simulink model "EV_Bus_Forward_before_noise_update"  (R2025a)
settings: Solver=ode23t  StartTime=0.0  StopTime=300  MaxStep=0.01  RelTol=1e-5  AbsTol=1e-7
model workspace (MAT data in the model file):
  Comp : object (value not decoded)
  MeasuredForceBias = 1114.3044183
  MeasuredTraction = [0 0.01 0.02 0.03 0.04 0.05 0.06 0.07 0.08 0.09 0.1 0.11 ... (60002 elements, 30001x2)]
  P : object (value not decoded)
  SignalNames : object (value not decoded)
  SlopeProfile = [0 85 100 140 155 180 200 300 0 0 4 4 ... (16 elements, 8x2)]
  SpeedProfile = [0 5 25 55 70 85 105 140 160 180 200 225 ... (32 elements, 16x2)]
  TemperatureProfile = [0  25; 150  30; 300  35]
values from neighbouring files (symbols this model uses):
  P =     [EV_Bus_parameters.mat]
symbols that are objects in the model workspace (value not decoded): Comp
(part 2 of 2)

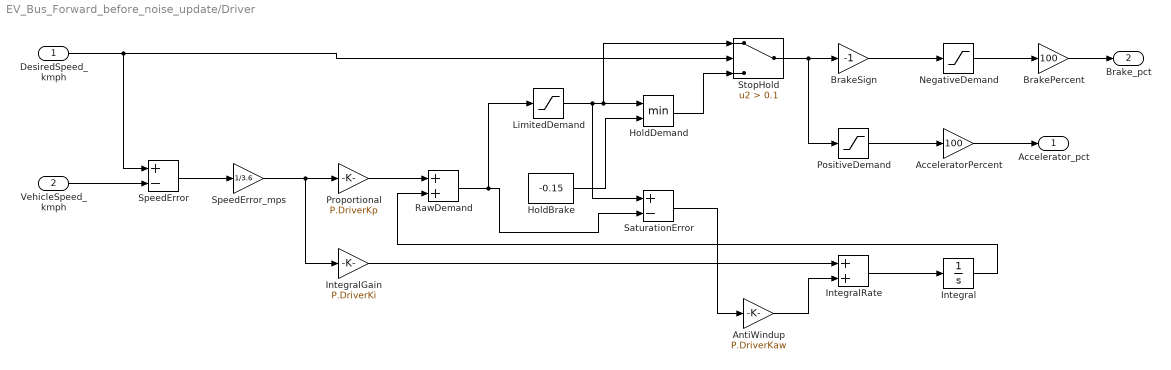
== system EV_Bus_Forward_before_noise_update/Driver ==
  DesiredSpeed_kmph : Inport
  VehicleSpeed_kmph : Inport  Port=2
  AcceleratorPercent : Gain  Gain=100
  AntiWindup : Gain  Gain=P.DriverKaw
  BrakePercent : Gain  Gain=100
  BrakeSign : Gain  Gain=-1
  HoldBrake : Constant  Value=-0.15
  HoldDemand : MinMax  Inputs=2
  Integral : Integrator  LimitOutput=on  UpperSaturationLimit=0.6  LowerSaturationLimit=-0.6
  IntegralGain : Gain  Gain=P.DriverKi
  IntegralRate : Sum
  LimitedDemand : Saturate  UpperLimit=1  LowerLimit=-1
  NegativeDemand : Saturate  UpperLimit=1  LowerLimit=0
  PositiveDemand : Saturate  UpperLimit=1  LowerLimit=0
  Proportional : Gain  Gain=P.DriverKp
  RawDemand : Sum
  SaturationError : Sum  Inputs=+-
  SpeedError : Sum  Inputs=+-
  SpeedError_mps : Gain  Gain=1/3.6
  StopHold : Switch  Criteria=u2 > Threshold  Threshold=0.1  SaturateOnIntegerOverflow=off  InputSameDT=off
  Accelerator_pct : Outport
  Brake_pct : Outport  Port=2
  wires:
  BrakePercent/1 -> Brake_pct/1
  NegativeDemand/1 -> BrakePercent/1
  BrakeSign/1 -> NegativeDemand/1
  AcceleratorPercent/1 -> Accelerator_pct/1
  PositiveDemand/1 -> AcceleratorPercent/1
  StopHold/1 -> PositiveDemand/1, BrakeSign/1
  HoldDemand/1 -> StopHold/3
  HoldBrake/1 -> HoldDemand/2
  IntegralRate/1 -> Integral/1
  AntiWindup/1 -> IntegralRate/2
  IntegralGain/1 -> IntegralRate/1
  SaturationError/1 -> AntiWindup/1
  LimitedDemand/1 -> HoldDemand/1, StopHold/1, SaturationError/1
  RawDemand/1 -> LimitedDemand/1, SaturationError/2
  Integral/1 -> RawDemand/2
  Proportional/1 -> RawDemand/1
  SpeedError_mps/1 -> Proportional/1, IntegralGain/1
  SpeedError/1 -> SpeedError_mps/1
  VehicleSpeed_kmph/1 -> SpeedError/2
  DesiredSpeed_kmph/1 -> SpeedError/1, StopHold/2

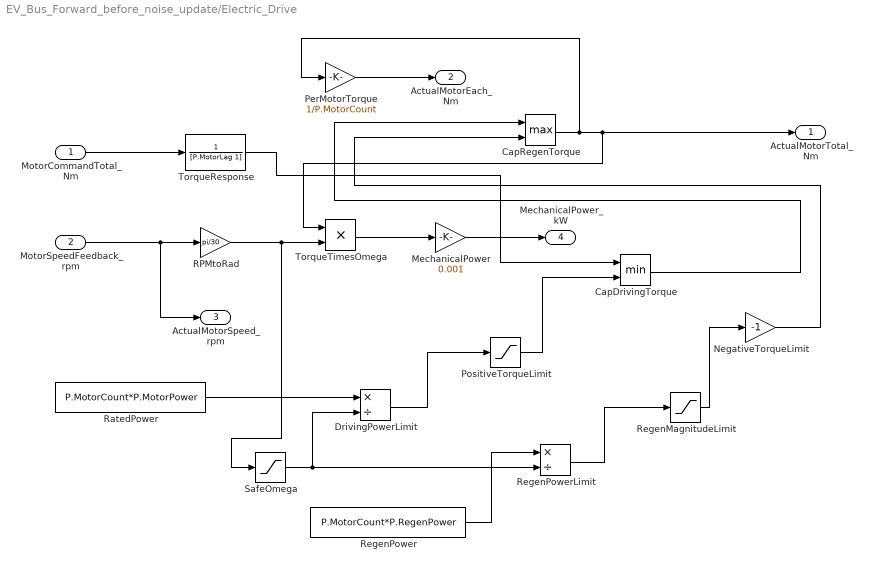
== system EV_Bus_Forward_before_noise_update/Electric_Drive ==
  MotorCommandTotal_Nm : Inport
  MotorSpeedFeedback_rpm : Inport  Port=2
  CapDrivingTorque : MinMax  Inputs=2
  CapRegenTorque : MinMax  Function=max  Inputs=2
  DrivingPowerLimit : Product  Inputs=*/
  MechanicalPower : Gain  Gain=0.001
  NegativeTorqueLimit : Gain  Gain=-1
  PerMotorTorque : Gain  Gain=1/P.MotorCount
  PositiveTorqueLimit : Saturate  UpperLimit=P.MotorCount*P.MotorPeakTorque  LowerLimit=0
  RPMtoRad : Gain  Gain=pi/30
  RatedPower : Constant  Value=P.MotorCount*P.MotorPower
  RegenMagnitudeLimit : Saturate  UpperLimit=P.MotorCount*P.RegenPeakTorque  LowerLimit=0
  RegenPower : Constant  Value=P.MotorCount*P.RegenPower
  RegenPowerLimit : Product  Inputs=*/
  SafeOmega : Saturate  UpperLimit=inf  LowerLimit=1
  TorqueResponse : TransferFcn  Denominator=[P.MotorLag 1]
  TorqueTimesOmega : Product  Inputs=**
  ActualMotorTotal_Nm : Outport
  ActualMotorEach_Nm : Outport  Port=2
  ActualMotorSpeed_rpm : Outport  Port=3
  MechanicalPower_kW : Outport  Port=4
  wires:
  MechanicalPower/1 -> MechanicalPower_kW/1
  TorqueTimesOmega/1 -> MechanicalPower/1
  MotorSpeedFeedback_rpm/1 -> ActualMotorSpeed_rpm/1, RPMtoRad/1
  PerMotorTorque/1 -> ActualMotorEach_Nm/1
  MotorCommandTotal_Nm/1 -> TorqueResponse/1
  CapRegenTorque/1 -> TorqueTimesOmega/1, ActualMotorTotal_Nm/1, PerMotorTorque/1
  NegativeTorqueLimit/1 -> CapRegenTorque/2
  CapDrivingTorque/1 -> CapRegenTorque/1
  PositiveTorqueLimit/1 -> CapDrivingTorque/2
  RegenMagnitudeLimit/1 -> NegativeTorqueLimit/1
  RegenPowerLimit/1 -> RegenMagnitudeLimit/1
  RegenPower/1 -> RegenPowerLimit/1
  DrivingPowerLimit/1 -> PositiveTorqueLimit/1
  SafeOmega/1 -> RegenPowerLimit/2, DrivingPowerLimit/2
  RatedPower/1 -> DrivingPowerLimit/1
  TorqueResponse/1 -> CapDrivingTorque/1
  RPMtoRad/1 -> SafeOmega/1, TorqueTimesOmega/2

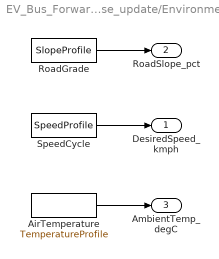
== system EV_Bus_Forward_before_noise_update/Environment ==
  AirTemperature : FromWorkspace  VariableName=TemperatureProfile
  RoadGrade : FromWorkspace  VariableName=SlopeProfile
  SpeedCycle : FromWorkspace  VariableName=SpeedProfile
  DesiredSpeed_kmph : Outport
  RoadSlope_pct : Outport  Port=2
  AmbientTemp_degC : Outport  Port=3
  wires:
  AirTemperature/1 -> AmbientTemp_degC/1
  RoadGrade/1 -> RoadSlope_pct/1
  SpeedCycle/1 -> DesiredSpeed_kmph/1

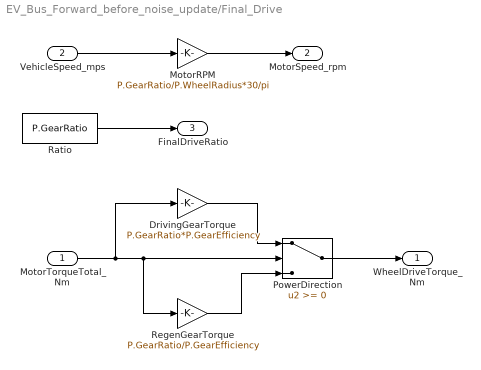
== system EV_Bus_Forward_before_noise_update/Final_Drive ==
  MotorTorqueTotal_Nm : Inport
  VehicleSpeed_mps : Inport  Port=2
  DrivingGearTorque : Gain  Gain=P.GearRatio*P.GearEfficiency
  MotorRPM : Gain  Gain=P.GearRatio/P.WheelRadius*30/pi
  PowerDirection : Switch  SaturateOnIntegerOverflow=off  InputSameDT=off
  Ratio : Constant  Value=P.GearRatio
  RegenGearTorque : Gain  Gain=P.GearRatio/P.GearEfficiency
  WheelDriveTorque_Nm : Outport
  MotorSpeed_rpm : Outport  Port=2
  FinalDriveRatio : Outport  Port=3
  wires:
  Ratio/1 -> FinalDriveRatio/1
  MotorRPM/1 -> MotorSpeed_rpm/1
  VehicleSpeed_mps/1 -> MotorRPM/1
  PowerDirection/1 -> WheelDriveTorque_Nm/1
  RegenGearTorque/1 -> PowerDirection/3
  DrivingGearTorque/1 -> PowerDirection/1
  MotorTorqueTotal_Nm/1 -> PowerDirection/2, RegenGearTorque/1, DrivingGearTorque/1

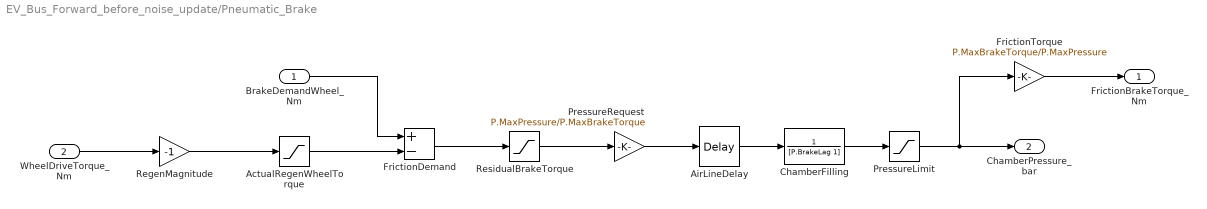
== system EV_Bus_Forward_before_noise_update/Pneumatic_Brake ==
  BrakeDemandWheel_Nm : Inport
  WheelDriveTorque_Nm : Inport  Port=2
  ActualRegenWheelTorque : Saturate  UpperLimit=inf  LowerLimit=0
  AirLineDelay : TransportDelay  DelayTime=P.BrakeDelay
  ChamberFilling : TransferFcn  Denominator=[P.BrakeLag 1]
  FrictionDemand : Sum  Inputs=+-
  FrictionTorque : Gain  Gain=P.MaxBrakeTorque/P.MaxPressure
  PressureLimit : Saturate  UpperLimit=P.MaxPressure  LowerLimit=0
  PressureRequest : Gain  Gain=P.MaxPressure/P.MaxBrakeTorque
  RegenMagnitude : Gain  Gain=-1
  ResidualBrakeTorque : Saturate  UpperLimit=P.MaxBrakeTorque  LowerLimit=0
  FrictionBrakeTorque_Nm : Outport
  ChamberPressure_bar : Outport  Port=2
  wires:
  FrictionTorque/1 -> FrictionBrakeTorque_Nm/1
  PressureLimit/1 -> ChamberPressure_bar/1, FrictionTorque/1
  ChamberFilling/1 -> PressureLimit/1
  AirLineDelay/1 -> ChamberFilling/1
  PressureRequest/1 -> AirLineDelay/1
  ResidualBrakeTorque/1 -> PressureRequest/1
  FrictionDemand/1 -> ResidualBrakeTorque/1
  ActualRegenWheelTorque/1 -> FrictionDemand/2
  BrakeDemandWheel_Nm/1 -> FrictionDemand/1
  RegenMagnitude/1 -> ActualRegenWheelTorque/1
  WheelDriveTorque_Nm/1 -> RegenMagnitude/1

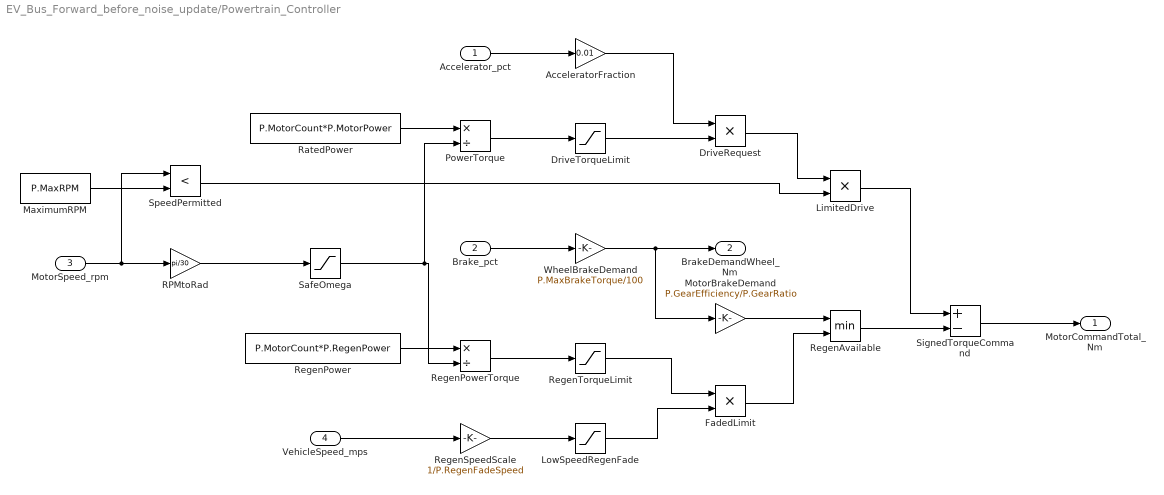
== system EV_Bus_Forward_before_noise_update/Powertrain_Controller ==
  Accelerator_pct : Inport
  Brake_pct : Inport  Port=2
  MotorSpeed_rpm : Inport  Port=3
  VehicleSpeed_mps : Inport  Port=4
  AcceleratorFraction : Gain  Gain=0.01
  DriveRequest : Product  Inputs=**
  DriveTorqueLimit : Saturate  UpperLimit=P.MotorCount*P.MotorPeakTorque  LowerLimit=0
  FadedLimit : Product  Inputs=**
  LimitedDrive : Product  Inputs=**
  LowSpeedRegenFade : Saturate  UpperLimit=1  LowerLimit=0
  MaximumRPM : Constant  Value=P.MaxRPM
  MotorBrakeDemand : Gain  Gain=P.GearEfficiency/P.GearRatio
  PowerTorque : Product  Inputs=*/
  RPMtoRad : Gain  Gain=pi/30
  RatedPower : Constant  Value=P.MotorCount*P.MotorPower
  RegenAvailable : MinMax  Inputs=2
  RegenPower : Constant  Value=P.MotorCount*P.RegenPower
  RegenPowerTorque : Product  Inputs=*/
  RegenSpeedScale : Gain  Gain=1/P.RegenFadeSpeed
  RegenTorqueLimit : Saturate  UpperLimit=P.MotorCount*P.RegenPeakTorque  LowerLimit=0
  SafeOmega : Saturate  UpperLimit=inf  LowerLimit=1
  SignedTorqueCommand : Sum  Inputs=+-
  SpeedPermitted : RelationalOperator  Operator=<  OutDataTypeStr=boolean  RndMeth=Simplest  InputSameDT=off
  WheelBrakeDemand : Gain  Gain=P.MaxBrakeTorque/100
  MotorCommandTotal_Nm : Outport
  BrakeDemandWheel_Nm : Outport  Port=2
  wires:
  SignedTorqueCommand/1 -> MotorCommandTotal_Nm/1
  RegenAvailable/1 -> SignedTorqueCommand/2
  LimitedDrive/1 -> SignedTorqueCommand/1
  SpeedPermitted/1 -> LimitedDrive/2
  DriveRequest/1 -> LimitedDrive/1
  FadedLimit/1 -> RegenAvailable/2
  LowSpeedRegenFade/1 -> FadedLimit/2
  RegenTorqueLimit/1 -> FadedLimit/1
  MotorBrakeDemand/1 -> RegenAvailable/1
  WheelBrakeDemand/1 -> BrakeDemandWheel_Nm/1, MotorBrakeDemand/1
  Brake_pct/1 -> WheelBrakeDemand/1
  MaximumRPM/1 -> SpeedPermitted/2
  DriveTorqueLimit/1 -> DriveRequest/2
  AcceleratorFraction/1 -> DriveRequest/1
  Accelerator_pct/1 -> AcceleratorFraction/1
  RegenSpeedScale/1 -> LowSpeedRegenFade/1
  VehicleSpeed_mps/1 -> RegenSpeedScale/1
  RegenPowerTorque/1 -> RegenTorqueLimit/1
  RegenPower/1 -> RegenPowerTorque/1
  PowerTorque/1 -> DriveTorqueLimit/1
  SafeOmega/1 -> PowerTorque/2, RegenPowerTorque/2
  RatedPower/1 -> PowerTorque/1
  RPMtoRad/1 -> SafeOmega/1
  MotorSpeed_rpm/1 -> SpeedPermitted/1, RPMtoRad/1

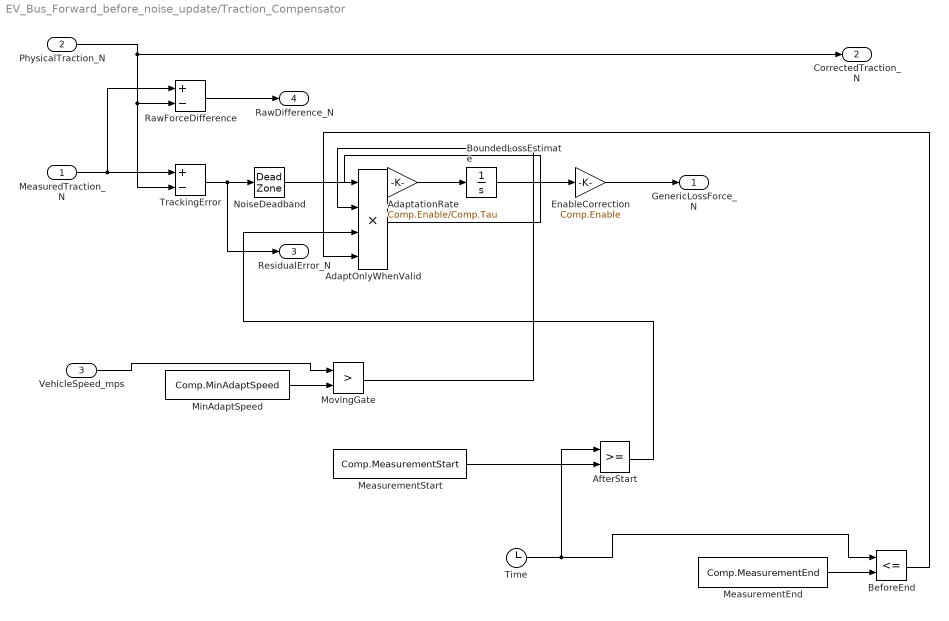
== system EV_Bus_Forward_before_noise_update/Traction_Compensator ==
  MeasuredTraction_N : Inport
  PhysicalTraction_N : Inport  Port=2
  VehicleSpeed_mps : Inport  Port=3
  AdaptOnlyWhenValid : Product  Inputs=****
  AdaptationRate : Gain  Gain=Comp.Enable/Comp.Tau
  AfterStart : RelationalOperator  OutDataTypeStr=boolean  RndMeth=Simplest  InputSameDT=off
  BeforeEnd : RelationalOperator  Operator=<=  OutDataTypeStr=boolean  RndMeth=Simplest  InputSameDT=off
  BoundedLossEstimate : Integrator  InitialCondition=Comp.InitialForce  LimitOutput=on  UpperSaturationLimit=Comp.Limit  LowerSaturationLimit=-Comp.Limit
  EnableCorrection : Gain  Gain=Comp.Enable
  MeasurementEnd : Constant  Value=Comp.MeasurementEnd
  MeasurementStart : Constant  Value=Comp.MeasurementStart
  MinAdaptSpeed : Constant  Value=Comp.MinAdaptSpeed
  MovingGate : RelationalOperator  Operator=>  OutDataTypeStr=boolean  RndMeth=Simplest  InputSameDT=off
  NoiseDeadband : DeadZone  LowerValue=-Comp.Deadband  UpperValue=Comp.Deadband
  RawForceDifference : Sum  Inputs=+-
  Time : Clock
  TrackingError : Sum  Inputs=+-
  GenericLossForce_N : Outport
  CorrectedTraction_N : Outport  Port=2
  ResidualError_N : Outport  Port=3
  RawDifference_N : Outport  Port=4
  wires:
  RawForceDifference/1 -> RawDifference_N/1
  MeasuredTraction_N/1 -> RawForceDifference/1, TrackingError/1
  PhysicalTraction_N/1 -> TrackingError/2, RawForceDifference/2, CorrectedTraction_N/1
  AdaptOnlyWhenValid/1 -> AdaptationRate/1
  BeforeEnd/1 -> AdaptOnlyWhenValid/4
  AfterStart/1 -> AdaptOnlyWhenValid/3
  MovingGate/1 -> AdaptOnlyWhenValid/2
  NoiseDeadband/1 -> AdaptOnlyWhenValid/1
  MeasurementEnd/1 -> BeforeEnd/2
  MeasurementStart/1 -> AfterStart/2
  Time/1 -> BeforeEnd/1, AfterStart/1
  MinAdaptSpeed/1 -> MovingGate/2
  VehicleSpeed_mps/1 -> MovingGate/1
  BoundedLossEstimate/1 -> EnableCorrection/1
  EnableCorrection/1 -> GenericLossForce_N/1
  TrackingError/1 -> NoiseDeadband/1, ResidualError_N/1
  AdaptationRate/1 -> BoundedLossEstimate/1

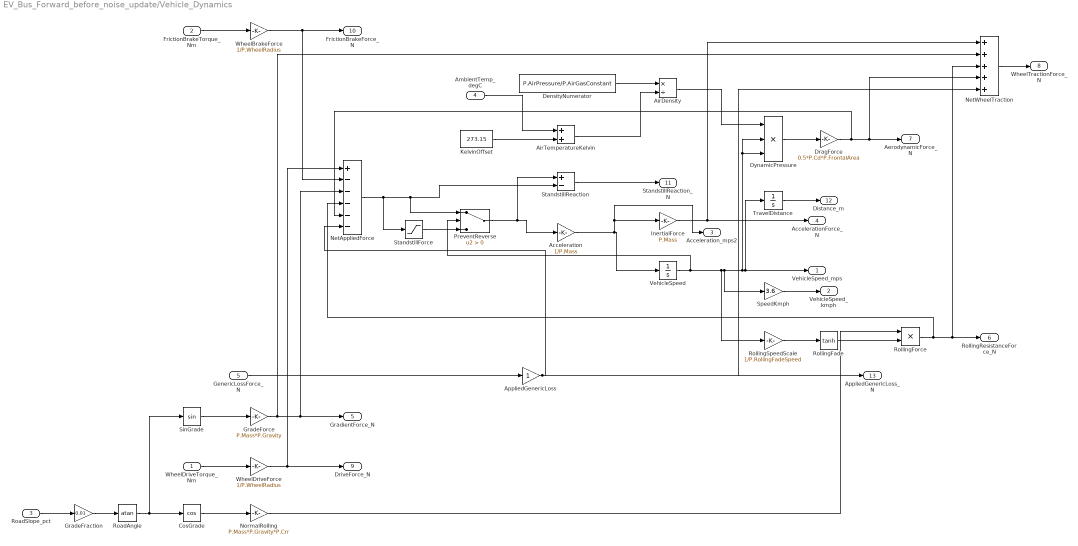
== system EV_Bus_Forward_before_noise_update/Vehicle_Dynamics ==
  WheelDriveTorque_Nm : Inport
  FrictionBrakeTorque_Nm : Inport  Port=2
  RoadSlope_pct : Inport  Port=3
  AmbientTemp_degC : Inport  Port=4
  GenericLossForce_N : Inport  Port=5
  Acceleration : Gain  Gain=1/P.Mass
  AirDensity : Product  Inputs=*/
  AirTemperatureKelvin : Sum
  AppliedGenericLoss : Gain
  CosGrade : Trigonometry  Operator=cos
  DensityNumerator : Constant  Value=P.AirPressure/P.AirGasConstant
  DragForce : Gain  Gain=0.5*P.Cd*P.FrontalArea
  DynamicPressure : Product  Inputs=***
  GradeForce : Gain  Gain=P.Mass*P.Gravity
  GradeFraction : Gain  Gain=0.01
  InertialForce : Gain  Gain=P.Mass
  KelvinOffset : Constant  Value=273.15
  NetAppliedForce : Sum  Inputs=+-----
  NetWheelTraction : Sum  Inputs=+++++
  NormalRolling : Gain  Gain=P.Mass*P.Gravity*P.Crr
  PreventReverse : Switch  Criteria=u2 > Threshold  SaturateOnIntegerOverflow=off  InputSameDT=off
  RoadAngle : Trigonometry  Operator=atan
  RollingFade : Trigonometry  Operator=tanh
  RollingForce : Product  Inputs=**
  RollingSpeedScale : Gain  Gain=1/P.RollingFadeSpeed
  SinGrade : Trigonometry
  SpeedKmph : Gain  Gain=3.6
  StandstillForce : Saturate  UpperLimit=inf  LowerLimit=0
  StandstillReaction : Sum  Inputs=+-
  TravelDistance : Integrator
  VehicleSpeed : Integrator  LimitOutput=on  LowerSaturationLimit=0
  WheelBrakeForce : Gain  Gain=1/P.WheelRadius
  WheelDriveForce : Gain  Gain=1/P.WheelRadius
  VehicleSpeed_mps : Outport
  VehicleSpeed_kmph : Outport  Port=2
  Acceleration_mps2 : Outport  Port=3
  AccelerationForce_N : Outport  Port=4
  GradientForce_N : Outport  Port=5
  RollingResistanceForce_N : Outport  Port=6
  AerodynamicForce_N : Outport  Port=7
  WheelTractionForce_N : Outport  Port=8
  DriveForce_N : Outport  Port=9
  FrictionBrakeForce_N : Outport  Port=10
  StandstillReaction_N : Outport  Port=11
  Distance_m : Outport  Port=12
  AppliedGenericLoss_N : Outport  Port=13
  wires:
  TravelDistance/1 -> Distance_m/1
  StandstillReaction/1 -> StandstillReaction_N/1
  NetWheelTraction/1 -> WheelTractionForce_N/1
  SpeedKmph/1 -> VehicleSpeed_kmph/1
  InertialForce/1 -> NetWheelTraction/1, AccelerationForce_N/1
  Acceleration/1 -> InertialForce/1, Acceleration_mps2/1, VehicleSpeed/1
  PreventReverse/1 -> Acceleration/1, StandstillReaction/1
  StandstillForce/1 -> PreventReverse/3
  NetAppliedForce/1 -> StandstillReaction/2, PreventReverse/1, StandstillForce/1
  DragForce/1 -> NetWheelTraction/4, AerodynamicForce_N/1, NetAppliedForce/5
  RollingForce/1 -> NetWheelTraction/3, RollingResistanceForce_N/1, NetAppliedForce/4
  GradeForce/1 -> NetAppliedForce/3, GradientForce_N/1, NetWheelTraction/2
  WheelBrakeForce/1 -> FrictionBrakeForce_N/1, NetAppliedForce/2
  WheelDriveForce/1 -> DriveForce_N/1, NetAppliedForce/1
  FrictionBrakeTorque_Nm/1 -> WheelBrakeForce/1
  WheelDriveTorque_Nm/1 -> WheelDriveForce/1
  DynamicPressure/1 -> DragForce/1
  AirDensity/1 -> DynamicPressure/1
  AirTemperatureKelvin/1 -> AirDensity/2
  DensityNumerator/1 -> AirDensity/1
  KelvinOffset/1 -> AirTemperatureKelvin/2
  AmbientTemp_degC/1 -> AirTemperatureKelvin/1
  RollingFade/1 -> RollingForce/2
  NormalRolling/1 -> RollingForce/1
  RollingSpeedScale/1 -> RollingFade/1
  VehicleSpeed/1 -> TravelDistance/1, VehicleSpeed_mps/1, DynamicPressure/2, DynamicPressure/3, SpeedKmph/1, RollingSpeedScale/1, PreventReverse/2
  CosGrade/1 -> NormalRolling/1
  SinGrade/1 -> GradeForce/1
  RoadAngle/1 -> SinGrade/1, CosGrade/1
  GradeFraction/1 -> RoadAngle/1
  RoadSlope_pct/1 -> GradeFraction/1
  AppliedGenericLoss/1 -> NetWheelTraction/5, NetAppliedForce/6, AppliedGenericLoss_N/1
  GenericLossForce_N/1 -> AppliedGenericLoss/1
